simulink model "flightControlSystem"  (R2026b)
settings: Solver=ode3  StopTime=TFinal
PreLoadFcn:
  | InitVars;
undefined symbols (not defined in the file or in its folder): control_power, feedforward_gains, integrator_limits, MC_PITCH_P, MC_PITCHRATE_D, MC_PITCHRATE_I, MC_PITCHRATE_MAX, MC_PITCHRATE_P, MC_ROLL_P, MC_ROLLRATE_D, MC_ROLLRATE_I, MC_ROLLRATE_MAX, MC_ROLLRATE_P, MC_YAW_P, MC_YAW_TQ_CUTOFF, MC_YAW_WEIGHT, MC_YAWRATE_D, MC_YAWRATE_I, MC_YAWRATE_MAX, MC_YAWRATE_P, MPC_ACC_DECOUPLE, MPC_LAND_ALT1, MPC_LAND_ALT2, MPC_LAND_ALT3, MPC_LAND_CRWL, MPC_LAND_SPEED, MPC_THR_HOVER, MPC_THR_MAX, MPC_THR_MIN, MPC_THR_XY_MARG, MPC_TILTMAX_AIR, MPC_VELD_LP, MPC_XY_P, MPC_XY_VEL_D_ACC, MPC_XY_VEL_I_ACC, MPC_XY_VEL_MAX, MPC_XY_VEL_P_ACC, MPC_Z_P, MPC_Z_VEL_D_ACC, MPC_Z_VEL_I_ACC, MPC_Z_VEL_MAX_DN, MPC_Z_VEL_MAX_UP, MPC_Z_VEL_P_ACC, SampleTime, timestamp
libraries: px4uORBlib x9, vrlib x8, aerolibutil x8, simulink x4, px4Utilslib x4, sharedutil x3, matrix_library x3, raspberrypiutilitieslib x2, px4Peripheralslib x2, sharedtransform x1, px4Sensorslib x1
(part 4 of 4)

== matlab function flightControlSystem/Estimator/Simulation Estimator/MATLAB Function6 ==
  data: roll input; qd output; pitch input; yaw input
function qd = eulerToQuaternion(roll, pitch, yaw)
    % Convert roll, pitch, yaw (in radians) to a quaternion
    cr = cos(roll / 2);
    sr = sin(roll / 2);
    cp = cos(pitch / 2);
    sp = sin(pitch / 2);
    cy = cos(yaw / 2);
    sy = sin(yaw / 2);

    qd = [cr * cp * cy + sr * sp * sy, ...
          sr * cp * cy - cr * sp * sy, ...
          cr * sp * cy + sr * cp * sy, ...
          cr * cp * sy - sr * sp * cy];
	qd = qd / norm(qd);
end

== matlab function flightControlSystem/Estimator/Simulation Estimator/MATLAB Function8 ==
  data: q_curr input; q_Delta output; q_prev input
function q_Delta = computeDeltaQuaternion(q_curr, q_prev)
% computeDeltaQuaternion - Computes the delta quaternion between two orientations
%
% Syntax: q_Delta = computeDeltaQuaternion(q_curr, q_prev)
%
% Inputs:
%   q_curr - current quaternion (1x4 vector or quaternion object)
%   q_prev - previous quaternion (1x4 vector or quaternion object)
%
% Output:
%   q_Delta - delta quaternion (1x4 vector)

% Ensure inputs are row vectors
q_curr = reshape(q_curr, 1, []);
q_prev = reshape(q_prev, 1, []);

% Compute the delta quaternion
q_Delta = quatmultiply(q_curr, quatinv(q_prev));

% Normalize the result
q_Delta = q_Delta / norm(q_Delta);
end

== matlab function flightControlSystem/Estimator/Estimator/set_vehicle_states_v116 ==
  data: x input; position output; y input; z input; vx input; vy input; vz input; heading input; xy_valid input; z_valid input; v_xy_valid input; v_z_valid input; dt input; MPC_VEL_NF_FRQ input; MPC_VEL_NF_BW input; MPC_VEL_LP input; MPC_VELD_LP input; velocity output; acceleration output; yaw output
function [position, velocity, acceleration, yaw] = set_vehicle_states_v116(x, y, z, vx, vy, vz, heading, xy_valid, z_valid, v_xy_valid, v_z_valid, dt, MPC_VEL_NF_FRQ, MPC_VEL_NF_BW, MPC_VEL_LP, MPC_VELD_LP)
%#codegen
% PX4 v1.16 set_vehicle_states — drop-in replacement for MATLAB Function5
% Reference: PX4-Autopilot/src/modules/mc_pos_control/MulticopterPositionControl.cpp
%
% v1.16 changes vs v1.14:
%   1. Velocity notch filter (removes frame vibration at MPC_VEL_NF_FRQ)
%   2. Velocity low-pass filter (MPC_VEL_LP Hz, smooths before D-term)
%   3. Derivative computed on LP-filtered signal (getState - prev_state)/dt
%   4. Derivative LP filter (MPC_VELD_LP Hz, same as v1.14 cutoff)
%
% AlphaFilter formula: tau=1/(2*pi*fc); alpha=dt/(dt+tau)
%   which equals: b=2*pi*fc*dt; a=b/(1+b) — same as v1.14 BlockLowPass

persistent notch_x1_xy notch_x2_xy notch_y1_xy notch_y2_xy
persistent notch_x1_z notch_x2_z notch_y1_z notch_y2_z
persistent vel_lp_state_xy vel_lp_state_z
persistent deriv_lp_state_x deriv_lp_state_y deriv_lp_state_z
persistent initialized

if isempty(initialized)
    notch_x1_xy = zeros(2,1); notch_x2_xy = zeros(2,1);
    notch_y1_xy = zeros(2,1); notch_y2_xy = zeros(2,1);
    notch_x1_z = 0; notch_x2_z = 0;
    notch_y1_z = 0; notch_y2_z = 0;
    vel_lp_state_xy = zeros(2,1);
    vel_lp_state_z = 0;
    deriv_lp_state_x = 0;
    deriv_lp_state_y = 0;
    deriv_lp_state_z = 0;
    initialized = true;
end

% Outputs
position = [x, y, z];
velocity = [vx, vy, vz];
acceleration = [0, 0, 0];
yaw = heading;

sample_freq = 1/dt;

% --- Notch filter coefficients (computed once, same for XY and Z) ---
if MPC_VEL_NF_FRQ > 0 && MPC_VEL_NF_BW > 0 && MPC_VEL_NF_FRQ < sample_freq/2
    alpha_n = tan(pi * MPC_VEL_NF_BW / sample_freq);
    beta_n = -cos(2*pi * MPC_VEL_NF_FRQ / sample_freq);
    a0_inv = 1 / (alpha_n + 1);
    b0 = a0_inv; b1_n = 2*beta_n*a0_inv; b2 = a0_inv;
    a1_n = b1_n; a2_n = (1 - alpha_n)*a0_inv;
    notch_enabled = true;
else
    b0=1; b1_n=0; b2=0; a1_n=0; a2_n=0;
    notch_enabled = false;
end

% --- LP filter alpha (velocity) ---
if MPC_VEL_LP > 0
    b_lp = 2*pi*MPC_VEL_LP*dt;
    alpha_lp = b_lp / (1 + b_lp);
    lp_enabled = true;
else
    alpha_lp = 1;
    lp_enabled = false;
end

% --- LP filter alpha (derivative) ---
b_d = 2*pi*MPC_VELD_LP*dt;
alpha_d = b_d / (1 + b_d);

% ============================================
% XY VELOCITY PROCESSING
% ============================================
velocity_xy = [vx; vy];

% Stage 1: Notch filter (PX4 NotchFilter::apply, Direct Form I)
if notch_enabled
    vel_notched_xy = b0*velocity_xy + b1_n*notch_x1_xy + b2*notch_x2_xy ...
                     - a1_n*notch_y1_xy - a2_n*notch_y2_xy;
    notch_x2_xy = notch_x1_xy; notch_x1_xy = velocity_xy;
    notch_y2_xy = notch_y1_xy; notch_y1_xy = vel_notched_xy;
else
    vel_notched_xy = velocity_xy;
end

% Stage 2: Velocity LP (PX4 AlphaFilter::update)
% _vel_xy_lp_filter.getState() — save BEFORE update
vel_xy_prev = vel_lp_state_xy;

if lp_enabled
    % state = state + alpha * (sample - state)
    vel_lp_state_xy = vel_lp_state_xy + alpha_lp * (vel_notched_xy - vel_lp_state_xy);
else
    vel_lp_state_xy = vel_notched_xy;
end

% states.velocity.xy() = _vel_xy_lp_filter.update(...)
velocity(1:2) = vel_lp_state_xy;

% Stage 3: Derivative LP (PX4 FilteredDerivative via AlphaFilter)
% deriv = (_vel_xy_lp_filter.getState() - vel_xy_prev) / dt_s
deriv_xy = (vel_lp_state_xy - vel_xy_prev) / dt;

% _vel_deriv_xy_lp_filter.update(deriv)
deriv_lp_state_x = deriv_lp_state_x + alpha_d * (deriv_xy(1) - deriv_lp_state_x);
deriv_lp_state_y = deriv_lp_state_y + alpha_d * (deriv_xy(2) - deriv_lp_state_y);
acceleration(1) = deriv_lp_state_x;
acceleration(2) = deriv_lp_state_y;

% ============================================
% Z VELOCITY PROCESSING
% ============================================

% Stage 1: Notch filter Z
if notch_enabled
    vel_notched_z = b0*vz + b1_n*notch_x1_z + b2*notch_x2_z ...
                    - a1_n*notch_y1_z - a2_n*notch_y2_z;
    notch_x2_z = notch_x1_z; notch_x1_z = vz;
    notch_y2_z = notch_y1_z; notch_y1_z = vel_notched_z;
else
    vel_notched_z = vz;
end

% Stage 2: Velocity LP Z
vel_z_prev = vel_lp_state_z;
if lp_enabled
    vel_lp_state_z = vel_lp_state_z + alpha_lp * (vel_notched_z - vel_lp_state_z);
else
    vel_lp_state_z = vel_notched_z;
end
velocity(3) = vel_lp_state_z;

% Stage 3: Derivative LP Z
deriv_z = (vel_lp_state_z - vel_z_prev) / dt;
deriv_lp_state_z = deriv_lp_state_z + alpha_d * (deriv_z - deriv_lp_state_z);
acceleration(3) = deriv_lp_state_z;
